simulink model "usv_openloop_3dof"  (R2024b)
settings: Solver=ode45  StartTime=0.0  StopTime=12  RelTol=1e-3
values from neighbouring files (symbols this model uses):
  tauN = tauList(k, 3)    [build_usv_openloop_3dof.m]
  tauX = tauList(k, 1)    [build_usv_openloop_3dof.m]
  tauY = tauList(k, 2)    [build_usv_openloop_3dof.m]
settings Model: Creator=qianr  LastModifiedBy=qianr
settings DataIOCC: SaveOutput=off

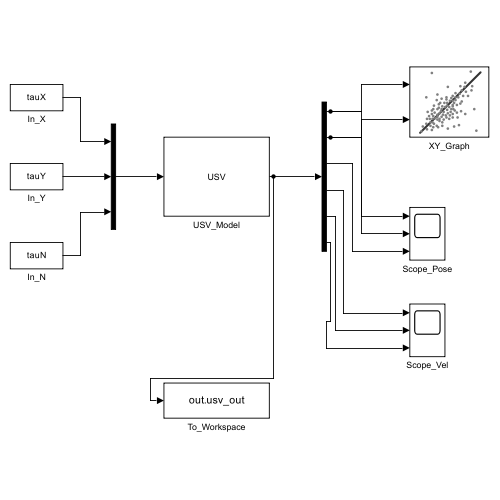
[thumbnail: Simulink's stored preview of the top-level diagram]
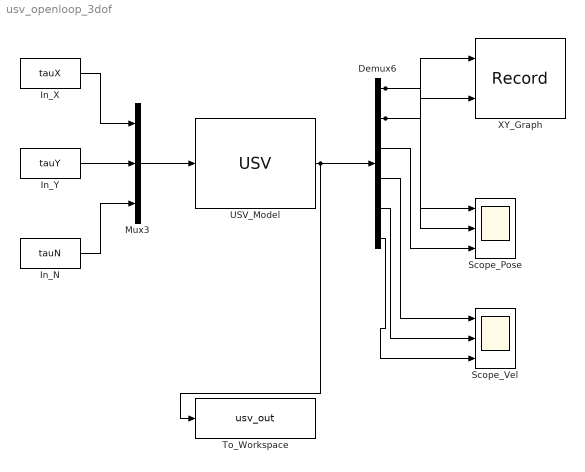
== system usv_openloop_3dof ==
  Demux6 : Demux  Outputs=6
  In_N : Constant  Value=tauN
  In_X : Constant  Value=tauX
  In_Y : Constant  Value=tauY
  Mux3 : Mux  Inputs=3
  Scope_Pose : Scope  NumInputPorts=3
  Scope_Vel : Scope  NumInputPorts=3
  To_Workspace : ToWorkspace  VariableName=usv_out  SampleTime=-1
  USV_Model : S-Function  FunctionName=USV  Parameters=cfg  SFunctionDeploymentMode=off  EnableBusSupport=off
  XY_Graph : Record  FileSettingsInternal="{\"entries\":[{\"content\":{\"excelSettings\":{\"content\":{},\"type\":\"Streamout.ExcelSettings\"}},\"type\":\"Streamout.FileSettingStorage\",\"uuid\":\"\"}],\"packageUris\":[\"http:\\/\\/schema.mathworks.com\\/mf0\\/streamout_blocks\\/R2020a\"],\"version\":\"1.0\"}"  Layout=[1 1]  SignalsInternal="{\"entries\":[{\"content\":{\"signals\":[{\"content\":{\"blockPath\":[],\"dimensions\":[1],\"domain\":\"\",\"lineColor\":\"#a2142f\",\"plots\":[ 1 ],\"port\":1,\"signalID\":1,\"signalName\":\"XY Graph:1\"},\"type\":\"RecordBlkView.Signal\",\"uuid\":\"\"},{\"content\":{\"blockPath\":[],\"dimensions\":[1],\"domain\":\"\",\"lineColor\":\"#139fff\",\"plots\":[ 1 ],\"port\":2,\"signalID\":2,\"signalName\":\"XY Graph:2\"},\"type\":\"RecordBlkView.Signal\",\"uuid\":\"\"}]},\"type\":\"RecordBlkView.InputSignals\",\"uuid\":\"\"}],\"packageUris\":[\"http:\\/\\/schema.mathworks.com\\/mf0\\/streamout_blocks\\/R2020a\"],\"version\":\"1.0\"}"  VisualizationBindings="{\"xyplotplugin\":{\"info\":[{\"series\":[{\"bindingParametersList\":[{\"parameter\":\"X-Axis\",\"signalID\":1,\"signalName\":\"XY Graph:1\"},{\"parameter\":\"Y-Axis\",\"signalID\":2,\"signalName\":\"XY Graph:2\"}],\"seriesID\":0}],\"subplotID\":1}]}}"  CompatibilityTag=XY
  wires:
  In_X/1 -> Mux3/1
  In_Y/1 -> Mux3/2
  In_N/1 -> Mux3/3
  Mux3/1 -> USV_Model/1
  USV_Model/1 -> Demux6/1, To_Workspace/1
  Demux6/1 -> XY_Graph/1, Scope_Pose/1
  Demux6/2 -> XY_Graph/2, Scope_Pose/2
  Demux6/3 -> Scope_Pose/3
  Demux6/4 -> Scope_Vel/1
  Demux6/5 -> Scope_Vel/2
  Demux6/6 -> Scope_Vel/3
